simulink model "ASM_Traffic_new"  (R2024a)
settings: Solver=ode1  StartTime=SIM.tstart.v  StopTime=SIM.tend.v  FixedStep=SIM.StepSize.v  RelTol=1e-3
PostLoadFcn:
  | if any(exist('dsrtsu_mdlpostloadfcn', 'file') ~= 0), dsrtsu_mdlpostloadfcn('Execute', bdroot); end
  | try, asm_mdl_postloadfcn(bdroot, 'UpdateModel', 3600); catch, disp(lasterr); end,
InitFcn:
  | , if any(exist('rtifpga_mdlclblib', 'file') ~= 0), rtifpga_mdlclblib('Init', bdroot); end,
  | , if any(exist('dsmpb_private', 'file') ~= 0), dsmpb_private('dsmpb_mdlclblib', 'Init', bdroot); end,
undefined symbols (not defined in the file): _to_, a0b2, ASM_BrakeHydraulics_DemoSystems, ASM_VehicleDynamics_DemoSystems, b98103fe8ad365046cd0, BrakeCircuit, CPT, Crankshaft, DiscIntNeverNeededParam, dsmsi, FinalDriveAssembly, MDL, ModeSignals, Pos_BrakePedal_Maneuver, rad, RefSignals, s_to_rpm, SIM, SoftECU, Suspension, Tire, Transmission
libraries: ASM_Traffic_lib x135, simulink x100, ASM_Utils_lib x77, ASM_VehicleDynamics_lib x70, ASM_Environment_lib x22, dsmpblib x20, dsmsilib x15, MDLD_Utils_lib x10, ASM_BrakeHydraulics_lib x3
(part 22 of 63)

== system ASM_Traffic_new/Engine/Interface_In/ModelSignals/Reset_States[0|1]_ ==
  In1 : Inport
  Gain : Gain  SaturateOnIntegerOverflow=on  OutDataTypeStr=Inherit: Same as input  ParamDataTypeStr=Inherit: Same as input
  Out1 : Outport  VectorParamsAs1DForOutWhenUnconnected=off
  wires:
  In1/1 -> Gain/1
  Gain/1 -> Out1/1

== system ASM_Traffic_new/Engine/Interface_In/ModelSignals/State_StartButton[-1|0|1|2]_ ==
  In1 : Inport
  Gain : Gain  SaturateOnIntegerOverflow=on  OutDataTypeStr=Inherit: Same as input  ParamDataTypeStr=Inherit: Same as input
  Out1 : Outport  VectorParamsAs1DForOutWhenUnconnected=off
  wires:
  Gain/1 -> Out1/1
  In1/1 -> Gain/1

== system ASM_Traffic_new/Engine/Interface_In/ModelSignals/Sw_CrankShaft_Reset[0Disabled|1Enabled]_ ==
  In1 : Inport
  Gain : Gain  SaturateOnIntegerOverflow=on  OutDataTypeStr=Inherit: Same as input  ParamDataTypeStr=Inherit: Same as input
  Out1 : Outport  VectorParamsAs1DForOutWhenUnconnected=off
  wires:
  In1/1 -> Gain/1
  Gain/1 -> Out1/1

== system ASM_Traffic_new/Engine/Interface_In/ModelSignals/Sw_Ignition[0Off|1On]_ ==
  In1 : Inport
  Gain : Gain  SaturateOnIntegerOverflow=on  OutDataTypeStr=Inherit: Same as input  ParamDataTypeStr=Inherit: Same as input
  Out1 : Outport  VectorParamsAs1DForOutWhenUnconnected=off
  wires:
  In1/1 -> Gain/1
  Gain/1 -> Out1/1

== system ASM_Traffic_new/Engine/Interface_In/ModelSignals/Sw_ModelDeskPlottingInterface[0Disabled|1Enabled]_ ==
  In1 : Inport
  Gain : Gain
  Out1 : Outport
  wires:
  Gain/1 -> Out1/1
  In1/1 -> Gain/1

== system ASM_Traffic_new/Engine/Interface_In/ModelSignals/Sw_ModelPortBlocks[0Disabled|1Enabled]_ ==
  In1 : Inport
  Gain : Gain
  Out1 : Outport
  wires:
  Gain/1 -> Out1/1
  In1/1 -> Gain/1

== system ASM_Traffic_new/Engine/Interface_In/ModelSignals/Sw_StarterReq[0Off|1On]_ ==
  In1 : Inport
  Gain : Gain  SaturateOnIntegerOverflow=on  OutDataTypeStr=Inherit: Same as input  ParamDataTypeStr=Inherit: Same as input
  Out1 : Outport  VectorParamsAs1DForOutWhenUnconnected=off
  wires:
  In1/1 -> Gain/1
  Gain/1 -> Out1/1

== system ASM_Traffic_new/Engine/Interface_In/ModelSignals/Trq_Decrease_Request_Fast_ESP[Nm]_ ==
  In1 : Inport
  Gain : Gain  SaturateOnIntegerOverflow=on  OutDataTypeStr=Inherit: Same as input  ParamDataTypeStr=Inherit: Same as input
  Out1 : Outport  VectorParamsAs1DForOutWhenUnconnected=off
  wires:
  In1/1 -> Gain/1
  Gain/1 -> Out1/1

== system ASM_Traffic_new/Engine/Interface_In/ModelSignals/Trq_Increase_Request_Fast_ESP[Nm]_ ==
  In1 : Inport
  Gain : Gain  SaturateOnIntegerOverflow=on  OutDataTypeStr=Inherit: Same as input  ParamDataTypeStr=Inherit: Same as input
  Out1 : Outport  VectorParamsAs1DForOutWhenUnconnected=off
  wires:
  In1/1 -> Gain/1
  Gain/1 -> Out1/1

== system ASM_Traffic_new/Engine/Interface_In/ModelSignals/Trq_Request_Extern1[Nm]_ ==
  In1 : Inport
  Gain : Gain  SaturateOnIntegerOverflow=on  OutDataTypeStr=Inherit: Same as input  ParamDataTypeStr=Inherit: Same as input
  Out1 : Outport  VectorParamsAs1DForOutWhenUnconnected=off
  wires:
  In1/1 -> Gain/1
  Gain/1 -> Out1/1

== system ASM_Traffic_new/Engine/Interface_In/ModelSignals/Trq_Request_Extern2[Nm]_ ==
  In1 : Inport
  Gain : Gain  SaturateOnIntegerOverflow=on  OutDataTypeStr=Inherit: Same as input  ParamDataTypeStr=Inherit: Same as input
  Out1 : Outport  VectorParamsAs1DForOutWhenUnconnected=off
  wires:
  In1/1 -> Gain/1
  Gain/1 -> Out1/1

== system ASM_Traffic_new/Engine/Interface_In/ModelSignals/Trq_Request_ICE[Nm]_ ==
  In1 : Inport
  Gain : Gain  SaturateOnIntegerOverflow=on  OutDataTypeStr=Inherit: Same as input  ParamDataTypeStr=Inherit: Same as input
  Out1 : Outport  VectorParamsAs1DForOutWhenUnconnected=off
  wires:
  In1/1 -> Gain/1
  Gain/1 -> Out1/1

== system ASM_Traffic_new/Engine/Interface_In/ModelSignals/Vehicle_Topology[-2|-1|0|2]_ ==
  In1 : Inport
  Gain : Gain  SaturateOnIntegerOverflow=on  OutDataTypeStr=Inherit: Same as input  ParamDataTypeStr=Inherit: Same as input
  Out1 : Outport  VectorParamsAs1DForOutWhenUnconnected=off
  wires:
  In1/1 -> Gain/1
  Gain/1 -> Out1/1

== system ASM_Traffic_new/Engine/Interface_In/ModelSignals/n_Engine[rpm]_ ==
  In1 : Inport
  Gain : Gain  SaturateOnIntegerOverflow=on  OutDataTypeStr=Inherit: Same as input  ParamDataTypeStr=Inherit: Same as input
  Out1 : Outport  VectorParamsAs1DForOutWhenUnconnected=off
  wires:
  In1/1 -> Gain/1
  Gain/1 -> Out1/1

== system ASM_Traffic_new/Engine/Interface_In/ModelSignals/n_Engine_Idle_Request[rpm]_ ==
  In1 : Inport
  Gain : Gain  SaturateOnIntegerOverflow=on  OutDataTypeStr=Inherit: Same as input  ParamDataTypeStr=Inherit: Same as input
  Out1 : Outport  VectorParamsAs1DForOutWhenUnconnected=off
  wires:
  In1/1 -> Gain/1
  Gain/1 -> Out1/1

== system ASM_Traffic_new/Engine/Interface_In/ModelSignals/v_x_Vehicle[km|h]_ ==
  In1 : Inport
  Gain : Gain  SaturateOnIntegerOverflow=on  OutDataTypeStr=Inherit: Same as input  ParamDataTypeStr=Inherit: Same as input
  Out1 : Outport  VectorParamsAs1DForOutWhenUnconnected=off
  wires:
  In1/1 -> Gain/1
  Gain/1 -> Out1/1

== system ASM_Traffic_new/Engine/Interface_Out/Control_ModelSignals/CrankAngle_Cyl[aTDC]_ ==
  In1 : Inport
  DummyGain : Gain  SaturateOnIntegerOverflow=on  OutDataTypeStr=Inherit: Same as input  ParamDataTypeStr=Inherit: Same as input
  Out1 : Outport  VectorParamsAs1DForOutWhenUnconnected=off
  wires:
  DummyGain/1 -> Out1/1
  In1/1 -> DummyGain/1

== system ASM_Traffic_new/Engine/Interface_Out/Control_ModelSignals/Enable_Trq_Shift_Request[0|1]_ ==
  In1 : Inport
  Gain : Gain  SaturateOnIntegerOverflow=on  OutDataTypeStr=Inherit: Same as input  ParamDataTypeStr=Inherit: Same as input
  Out1 : Outport  VectorParamsAs1DForOutWhenUnconnected=off
  wires:
  Gain/1 -> Out1/1
  In1/1 -> Gain/1

== system ASM_Traffic_new/Engine/Interface_Out/Control_ModelSignals/EngOP_Num[]_ ==
  In1 : Inport
  DummyGain : Gain  SaturateOnIntegerOverflow=on  OutDataTypeStr=Inherit: Same as input  ParamDataTypeStr=Inherit: Same as input
  Out1 : Outport  VectorParamsAs1DForOutWhenUnconnected=off
  wires:
  In1/1 -> DummyGain/1
  DummyGain/1 -> Out1/1

== system ASM_Traffic_new/Engine/Interface_Out/Control_ModelSignals/Pos_AccPedal_Meas[%]_ ==
  In1 : Inport
  DummyGain : Gain  SaturateOnIntegerOverflow=on  OutDataTypeStr=Inherit: Same as input  ParamDataTypeStr=Inherit: Same as input
  Out1 : Outport  VectorParamsAs1DForOutWhenUnconnected=off
  wires:
  DummyGain/1 -> Out1/1
  In1/1 -> DummyGain/1

== system ASM_Traffic_new/Engine/Interface_Out/Control_ModelSignals/State_ICEngine[0|1|2|3|4]_ ==
  In1 : Inport
  Gain : Gain  SaturateOnIntegerOverflow=on  OutDataTypeStr=Inherit: Same as input  ParamDataTypeStr=Inherit: Same as input
  Out1 : Outport  VectorParamsAs1DForOutWhenUnconnected=off
  wires:
  In1/1 -> Gain/1
  Gain/1 -> Out1/1

== system ASM_Traffic_new/Engine/Interface_Out/Control_ModelSignals/State_StartStop[1Off|2NotReady|3Ready|4EngStopped]_ ==
  In1 : Inport
  Gain : Gain  SaturateOnIntegerOverflow=on  OutDataTypeStr=Inherit: Same as input  ParamDataTypeStr=Inherit: Same as input
  Out1 : Outport  VectorParamsAs1DForOutWhenUnconnected=off
  wires:
  In1/1 -> Gain/1
  Gain/1 -> Out1/1

== system ASM_Traffic_new/Engine/Interface_Out/Control_ModelSignals/Sw_Replace_Env[0|1]_ ==
  In1 : Inport
  DummyGain : Gain  SaturateOnIntegerOverflow=on  OutDataTypeStr=Inherit: Same as input  ParamDataTypeStr=Inherit: Same as input
  Out1 : Outport  VectorParamsAs1DForOutWhenUnconnected=off
  wires:
  DummyGain/1 -> Out1/1
  In1/1 -> DummyGain/1

== system ASM_Traffic_new/Engine/Interface_Out/Control_ModelSignals/Sw_Starter[0Off|1On]_ ==
  In1 : Inport
  Gain : Gain  SaturateOnIntegerOverflow=on  OutDataTypeStr=Inherit: Same as input  ParamDataTypeStr=Inherit: Same as input
  Out1 : Outport  VectorParamsAs1DForOutWhenUnconnected=off
  wires:
  In1/1 -> Gain/1
  Gain/1 -> Out1/1

== system ASM_Traffic_new/Engine/Interface_Out/Control_ModelSignals/T_Ambient[degC]_ ==
  In1 : Inport
  DummyGain : Gain  SaturateOnIntegerOverflow=on  OutDataTypeStr=Inherit: Same as input  ParamDataTypeStr=Inherit: Same as input
  Out1 : Outport  VectorParamsAs1DForOutWhenUnconnected=off
  wires:
  DummyGain/1 -> Out1/1
  In1/1 -> DummyGain/1

== system ASM_Traffic_new/Engine/Interface_Out/Control_ModelSignals/Trq_MeanEff_Engine_Meas[Nm]_ ==
  In1 : Inport
  DummyGain : Gain  SaturateOnIntegerOverflow=on  OutDataTypeStr=Inherit: Same as input  ParamDataTypeStr=Inherit: Same as input
  Out1 : Outport  VectorParamsAs1DForOutWhenUnconnected=off
  wires:
  DummyGain/1 -> Out1/1
  In1/1 -> DummyGain/1

== system ASM_Traffic_new/Engine/Interface_Out/Control_ModelSignals/Trq_Shift_Request[Nm]_ ==
  In1 : Inport
  Gain : Gain  SaturateOnIntegerOverflow=on  OutDataTypeStr=Inherit: Same as input  ParamDataTypeStr=Inherit: Same as input
  Out1 : Outport  VectorParamsAs1DForOutWhenUnconnected=off
  wires:
  In1/1 -> Gain/1
  Gain/1 -> Out1/1

== system ASM_Traffic_new/Engine/Interface_Out/Control_ModelSignals/n_Engine_Idle_Set[rpm]_ ==
  In1 : Inport
  Gain : Gain  SaturateOnIntegerOverflow=on  OutDataTypeStr=Inherit: Same as input  ParamDataTypeStr=Inherit: Same as input
  Out1 : Outport  VectorParamsAs1DForOutWhenUnconnected=off
  wires:
  In1/1 -> Gain/1
  Gain/1 -> Out1/1

== system ASM_Traffic_new/Engine/Interface_Out/Control_ModelSignals/n_Engine_Meas[rpm]_ ==
  In1 : Inport
  DummyGain : Gain  SaturateOnIntegerOverflow=on  OutDataTypeStr=Inherit: Same as input  ParamDataTypeStr=Inherit: Same as input
  Out1 : Outport  VectorParamsAs1DForOutWhenUnconnected=off
  wires:
  In1/1 -> DummyGain/1
  DummyGain/1 -> Out1/1

== system ASM_Traffic_new/Engine/Interface_Out/Control_ModelSignals/p_Ambient[Pa]_ ==
  In1 : Inport
  DummyGain : Gain  SaturateOnIntegerOverflow=on  OutDataTypeStr=Inherit: Same as input  ParamDataTypeStr=Inherit: Same as input
  Out1 : Outport  VectorParamsAs1DForOutWhenUnconnected=off
  wires:
  In1/1 -> DummyGain/1
  DummyGain/1 -> Out1/1

== system ASM_Traffic_new/Engine/Interface_Out/Plant_ModelSignals/T_Coolant_ICE[degC]_ ==
  In1 : Inport
  Gain : Gain  SaturateOnIntegerOverflow=on  OutDataTypeStr=Inherit: Same as input  ParamDataTypeStr=Inherit: Same as input
  Out1 : Outport  VectorParamsAs1DForOutWhenUnconnected=off
  wires:
  Gain/1 -> Out1/1
  In1/1 -> Gain/1

== system ASM_Traffic_new/Engine/Interface_Out/Plant_ModelSignals/Trq_Fric_Engine[Nm]_ ==
  In1 : Inport
  Gain : Gain  SaturateOnIntegerOverflow=on  OutDataTypeStr=Inherit: Same as input  ParamDataTypeStr=Inherit: Same as input
  Out1 : Outport  VectorParamsAs1DForOutWhenUnconnected=off
  wires:
  In1/1 -> Gain/1
  Gain/1 -> Out1/1

== system ASM_Traffic_new/Engine/Interface_Out/Plant_ModelSignals/Trq_MeanEff_Engine[Nm]_ ==
  In1 : Inport
  Gain : Gain  SaturateOnIntegerOverflow=on  OutDataTypeStr=Inherit: Same as input  ParamDataTypeStr=Inherit: Same as input
  Out1 : Outport  VectorParamsAs1DForOutWhenUnconnected=off
  wires:
  In1/1 -> Gain/1
  Gain/1 -> Out1/1

== system ASM_Traffic_new/Engine/Interface_Out/Plant_ModelSignals/Type_Engine[0Unkown|1Other|2Otto|3Diesel|4Electric]_ ==
  In1 : Inport
  DummyGain : Gain  SaturateOnIntegerOverflow=on  OutDataTypeStr=Inherit: Same as input  ParamDataTypeStr=Inherit: Same as input
  Out1 : Outport  VectorParamsAs1DForOutWhenUnconnected=off
  wires:
  In1/1 -> DummyGain/1
  DummyGain/1 -> Out1/1

== system ASM_Traffic_new/Engine/Plant/EngineBasic/ASMSignalCollector ==
  BusCreator : BusCreator  Inputs=2
  ASMSIgnalBus : Outport  VectorParamsAs1DForOutWhenUnconnected=off
  wires:
  [ASMBUS_FUEL_CONSUMPTION] -> BusCreator/2
  BusCreator/1 -> ASMSIgnalBus/1  "Plant"
  [ASMBUS_ENGINE] -> BusCreator/1

== system ASM_Traffic_new/Engine/Plant/UserInterface/ASMSignalBus_Plant ==
  In : Inport
  Terminator_1 : Terminator
  tag scope: ASMBUS_Engine_Plant=global
  wires:
  [ASMBUS_Engine_Plant] -> Terminator_1/1
  In/1 -> [ASMBUS_Engine_Plant]  "Plant"

== system ASM_Traffic_new/Engine/Plant/UserInterface/DISP_Plant ==
  note: Dummy blocks for ControlDesk layout.
      | Might be replaced when simulating virtual vehicles.
  Interface_In : Inport
  In : Inport  Port=2
  Bus Selector1 : BusSelector  OutputSignals=Engine.Trq_Eff_Engine[Nm],Engine.Trq_Fric_Engine[Nm],Engine.Trq_Ind_Engine[Nm]
  Bus Selector10 : BusSelector  OutputSignals=FuelConsumption.CO2_Emission.CO2_Emission[kg|h],FuelConsumption.CO2_Emission.CO2_Emission_Total[kg],FuelConsumption.Fuel_Consumption[l|h],FuelConsumption.Fuel_Consumption_Total[l],FuelConsumption.mdot_Fuel[g|h],FuelConsumption.b_e[g|kWh],FuelConsumption.Efficiency.eta_Eff_Engine[0_1],FuelConsumption.Efficiency.eta_Ind_Engine[0_1],FuelConsumption.Efficiency.eta_Mechanical_Engine[0_1]
  Bus Selector2 : BusSelector  OutputSignals=ExternalModel.v_x_Vehicle[km|h]
  CO2_Emission[kg|100km] : Subsystem
      mask Display: disp('')
  CO2_Emission[kg|100km]_ : Subsystem
  CO2_Emission[kg|h] : Subsystem
      mask Display: disp('')
  CO2_Emission_Total[kg] : Subsystem
      mask Display: disp('')
  CarbonEmission : Scope  NumInputPorts=3
  Efficiency : Scope  NumInputPorts=3
  Engine : Scope  NumInputPorts=3
  FuelConsumption : Scope  NumInputPorts=5
  FuelTank : Constant  Value=0.5
  FuelTank[0|1] : Subsystem
      mask Display: disp('')
  Fuel_Consumption[L|100km] : Subsystem
      mask Display: disp('')
  Fuel_Consumption[L|100km]_ : Subsystem
  Fuel_Consumption[l|h] : Subsystem
      mask Display: disp('')
  Fuel_Consumption_Total[l] : Subsystem
      mask Display: disp('')
  T_Water : Constant
  T_Water[degC] : Subsystem
      mask Display: disp('')
  Terminator : Terminator
  Terminator2 : Terminator
  Trq_Eff_Engine[Nm] : Subsystem
      mask Display: disp('')
  Trq_Fric_Engine[Nm] : Subsystem
      mask Display: disp('')
  Trq_Ind_Engine[Nm] : Subsystem
      mask Display: disp('')
  b_e[g|kWh] : Subsystem
      mask Display: disp('')
  eta_Eff_Engine[0_1] : Subsystem
      mask Display: disp('')
  eta_Ind_Engine[0_1] : Subsystem
      mask Display: disp('')
  eta_Mechanical_Engine[0_1] : Subsystem
      mask Display: disp('')
  mdot_Fuel[g|h] : Subsystem
      mask Display: disp('')
  wires:
  Bus Selector2/1 -> CO2_Emission[kg|100km]_/1(v_Vehicle[km|h]), Fuel_Consumption[L|100km]_/1(v_Vehicle[km|h])  "<v_x_Vehicle[km|h]>"
  Interface_In/1 -> Bus Selector2/1
  Bus Selector10/4 -> Fuel_Consumption_Total[l]/1(In1)  "<Fuel_Consumption_Total[l]>"
  T_Water[degC]/1(Out1) -> Terminator2/1
  FuelTank/1 -> FuelTank[0|1]/1(In1)
  Fuel_Consumption[L|100km]/1(Out1) -> FuelConsumption/1  "Fuel_Conumption[l|100km]"
  T_Water/1 -> T_Water[degC]/1(In1)
  FuelTank[0|1]/1(Out1) -> Terminator/1
  Trq_Ind_Engine[Nm]/1(Out1) -> Engine/3  "Trq_Ind_Engine[Nm]"
  Bus Selector1/1 -> Trq_Eff_Engine[Nm]/1(In1)  "<Trq_Eff_Engine[Nm]>"
  Fuel_Consumption[L|100km]_/1(Fuel_Consumption[L|100km]) -> Fuel_Consumption[L|100km]/1(In1)
  Bus Selector1/3 -> Trq_Ind_Engine[Nm]/1(In1)  "<Trq_Ind_Engine[Nm]>"
  Trq_Fric_Engine[Nm]/1(Out1) -> Engine/2  "Trq_Fric_Engine[Nm]"
  CO2_Emission_Total[kg]/1(Out1) -> CarbonEmission/3  "CO2_Emission_Total[kg]"
  Bus Selector10/3 -> Fuel_Consumption[l|h]/1(In1), Fuel_Consumption[L|100km]_/2(Fuel_Consumption[l|h])  "<Fuel_Consumption[l|h]>"
  Bus Selector1/2 -> Trq_Fric_Engine[Nm]/1(In1)  "<Trq_Fric_Engine[Nm]>"
  CO2_Emission[kg|100km]_/1(CO2_Emission[kg|100km]) -> CO2_Emission[kg|100km]/1(In1)
  eta_Eff_Engine[0_1]/1(Out1) -> Efficiency/1  "eta_Eff_Engine[0_1]"
  Bus Selector10/5 -> mdot_Fuel[g|h]/1(In1)  "<mdot_Fuel[g|h]>"
  Bus Selector10/1 -> CO2_Emission[kg|h]/1(In1), CO2_Emission[kg|100km]_/2(CO2_Emission[kg|h])  "<CO2_Emission[kg|h]>"
  Bus Selector10/6 -> b_e[g|kWh]/1(In1)  "<b_e[g|kWh]>"
  Bus Selector10/2 -> CO2_Emission_Total[kg]/1(In1)  "<CO2_Emission_Total[kg]>"
  Trq_Eff_Engine[Nm]/1(Out1) -> Engine/1  "Trq_Eff_Engine[Nm]"
  CO2_Emission[kg|h]/1(Out1) -> CarbonEmission/2  "CO2_Emission[kg|h]"
  Bus Selector10/7 -> eta_Eff_Engine[0_1]/1(In1)  "<eta_Eff_Engine[0_1]>"
  Fuel_Consumption_Total[l]/1(Out1) -> FuelConsumption/3  "Fuel_Consumption_Total[l]"
  Bus Selector10/9 -> eta_Mechanical_Engine[0_1]/1(In1)  "<eta_Mechanical_Engine[0_1]>"
  In/1 -> Bus Selector1/1, Bus Selector10/1
  Fuel_Consumption[l|h]/1(Out1) -> FuelConsumption/2  "Fuel_Consumption[l|h]"
  eta_Mechanical_Engine[0_1]/1(Out1) -> Efficiency/3  "eta_Mechanical_Engine[0_1]"
  Bus Selector10/8 -> eta_Ind_Engine[0_1]/1(In1)  "<eta_Ind_Engine[0_1]>"
  eta_Ind_Engine[0_1]/1(Out1) -> Efficiency/2  "eta_Ind_Engine[0_1]"
  CO2_Emission[kg|100km]/1(Out1) -> CarbonEmission/1  "CO2_Emission[kg|100km]"
  b_e[g|kWh]/1(Out1) -> FuelConsumption/5  "b_e[g|kWh]"
  mdot_Fuel[g|h]/1(Out1) -> FuelConsumption/4  "mdot_Fuel[g|h]"

== system ASM_Traffic_new/Engine/Plant/UserInterface/PAR_Plant ==
  Termination : Constant  Value=0
  Out : Outport  VectorParamsAs1DForOutWhenUnconnected=off
  wires:
  Termination/1 -> Out/1

== system ASM_Traffic_new/Engine/SignalInterface/ASMSignalInterface/signal_structure ==
  ASMSignalBus : Inport
  BusSelector_1 : BusSelector  OutputSignals=Control,Plant
  CO2_Emission : BusSelector  OutputSignals=CO2_Emission[kg|h],CO2_Emission_Total[kg]
  ContentID : Constant  Value=278498219
  Control : BusSelector  OutputSignals=ESP_Fast_Torque_Set,Shift_Torque_Set,Torque_Intervention,IdleSpeedControl,EngineOperation
  DataTypeConversion_2 : DataTypeConversion  OutDataTypeStr=double
  ESP_Fast_Torque_Set : BusSelector  OutputSignals=Sw_Engine_Dynamics_Fast[0|1],Enable_Trq_Request_Fast[0|1],Trq_Request_Fast[Nm]
  Efficiency : BusSelector  OutputSignals=eta_Eff_Engine[0_1],eta_Ind_Engine[0_1],eta_Mechanical_Engine[0_1]
  Engine : BusSelector  OutputSignals=TimeConst_Engine_Dynamics[s],Trq_Eff_Engine[Nm],Trq_Driver_Des[Nm],Trq_FullLoad_Engine[Nm],Trq_Fric_Engine[Nm],Trq_Ind_Engine[Nm],Trq_Driver_Ind_Des[Nm],Trq_Engine_Ind_Max[Nm]
  EngineOperation : BusSelector  OutputSignals=State_Engine[0|1|2|3|4],Sw_Starter[0Off|1On]
  FuelConsumption : BusSelector  OutputSignals=mdot_Fuel[g|h],b_e[g|kWh],Efficiency,CO2_Emission,Fuel_Consumption[l|h],Fuel_Consumption_Total[l]
  IdleSpeedControl : BusSelector  OutputSignals=n_Engine_Idle_Set[rpm],Pos_AccPedal_Ctrl[%]
  InfoBlock : Subsystem
      mask Display: fprintf('Structural changes of the signal bus require an update \nof the ''ASMSignalCollector'' block. \n\nTo start the update process double click the parent block.\n\n WARNING:\n During update this subsystem will be cleared completely')
  MDLD_DATA_CAPTURE : MDLD_Utils_lib/ModelDeskPlotInterface/DataCapture_Sfcn/MDLD_DATA_CAPTURE  inputPortWidth=41  measurementSignals=[0 0 0 0 0 0 0 0 0 0 0 0 0 0 0 0 0 0 0 0 0 0 0 0 0 0 0 0 0 0 0 0 0 0 0 0 0 0 0 0 0]  downsampling=1  samplingPeriod=SIM.StepSize.v  uuid=0  ASMProperties=struct('Name','mdld_data_capture','Version','1.0','Library','mdld_utils_lib')  startTriggerDelay=0  startTriggerLogic=0  startTriggerCount=0  startTriggerConditions=[0,0,0,0,0,0,0,0,0]  stopTriggerDelay=0  stopTriggerLogic=0  stopTriggerCount=0  stopTriggerConditions=[0,0,0,0,0,0,0,0,0]  ContentID_RefStruct=278498219
  Plant : BusSelector  OutputSignals=Engine,FuelConsumption
  Shift_Torque_Set : BusSelector  OutputSignals=Trq_Driver_Ind_Des[Nm],Trq_Ind_Set[Nm],Enable_Trq_Ind_Set[0|1]
  SignalFilter : Mux  Inputs=41
  SignalFilterGain : Gain
  Terminator : Terminator
  Torque_Intervention : BusSelector  OutputSignals=Pos_AccPedal_Request[%],Enable_Trq_Request_Fast[0|1],Enable_Trq_Request_Extern1[0|1],Enable_Trq_Request_Extern2[0|1],Enable_Trq_Request_Extern3[0|1],Trq_Request_Fast[Nm],Trq_Request_Extern1[Nm],Trq_Request_Extern2[Nm],Trq_Request_Extern3[Nm],Pos_AccPedal_Request_Fast[%],Pos_AccPedal_Request_Extern1[%],Pos_AccPedal_Request_Extern2[%],Pos_AccPedal_Request_Extern3[%],Pos_AccPedal_Request_Driver[%]
  wires:
  ASMSignalBus/1 -> BusSelector_1/1
  BusSelector_1/1 -> Control/1  "<Control>"
  Control/1 -> ESP_Fast_Torque_Set/1  "<ESP_Fast_Torque_Set>"
  Control/2 -> Shift_Torque_Set/1  "<Shift_Torque_Set>"
  Control/3 -> Torque_Intervention/1  "<Torque_Intervention>"
  Control/4 -> IdleSpeedControl/1  "<IdleSpeedControl>"
  Control/5 -> EngineOperation/1  "<EngineOperation>"
  BusSelector_1/2 -> Plant/1  "<Plant>"
  Plant/1 -> Engine/1  "<Engine>"
  Plant/2 -> FuelConsumption/1  "<FuelConsumption>"
  FuelConsumption/3 -> Efficiency/1  "<Efficiency>"
  FuelConsumption/4 -> CO2_Emission/1  "<CO2_Emission>"
  ContentID/1 -> Terminator/1
  ESP_Fast_Torque_Set/1 -> SignalFilter/1  "<Sw_Engine_Dynamics_Fast[0|1]>"
  ESP_Fast_Torque_Set/2 -> DataTypeConversion_2/1  "<Enable_Trq_Request_Fast[0|1]>"
  DataTypeConversion_2/1 -> SignalFilter/2
  ESP_Fast_Torque_Set/3 -> SignalFilter/3  "<Trq_Request_Fast[Nm]>"
  Shift_Torque_Set/1 -> SignalFilter/4  "<Trq_Driver_Ind_Des[Nm]>"
  Shift_Torque_Set/2 -> SignalFilter/5  "<Trq_Ind_Set[Nm]>"
  Shift_Torque_Set/3 -> SignalFilter/6  "<Enable_Trq_Ind_Set[0|1]>"
  Torque_Intervention/1 -> SignalFilter/7  "<Pos_AccPedal_Request[%]>"
  Torque_Intervention/2 -> SignalFilter/8  "<Enable_Trq_Request_Fast[0|1]>"
  Torque_Intervention/3 -> SignalFilter/9  "<Enable_Trq_Request_Extern1[0|1]>"
  Torque_Intervention/4 -> SignalFilter/10  "<Enable_Trq_Request_Extern2[0|1]>"
  Torque_Intervention/5 -> SignalFilter/11  "<Enable_Trq_Request_Extern3[0|1]>"
  Torque_Intervention/6 -> SignalFilter/12  "<Trq_Request_Fast[Nm]>"
  Torque_Intervention/7 -> SignalFilter/13  "<Trq_Request_Extern1[Nm]>"
  Torque_Intervention/8 -> SignalFilter/14  "<Trq_Request_Extern2[Nm]>"
  Torque_Intervention/9 -> SignalFilter/15  "<Trq_Request_Extern3[Nm]>"
  Torque_Intervention/10 -> SignalFilter/16  "<Pos_AccPedal_Request_Fast[%]>"
  Torque_Intervention/11 -> SignalFilter/17  "<Pos_AccPedal_Request_Extern1[%]>"
  Torque_Intervention/12 -> SignalFilter/18  "<Pos_AccPedal_Request_Extern2[%]>"
  Torque_Intervention/13 -> SignalFilter/19  "<Pos_AccPedal_Request_Extern3[%]>"
  Torque_Intervention/14 -> SignalFilter/20  "<Pos_AccPedal_Request_Driver[%]>"
  IdleSpeedControl/1 -> SignalFilter/21  "<n_Engine_Idle_Set[rpm]>"
  IdleSpeedControl/2 -> SignalFilter/22  "<Pos_AccPedal_Ctrl[%]>"
  EngineOperation/1 -> SignalFilter/23  "<State_Engine[0|1|2|3|4]>"
  EngineOperation/2 -> SignalFilter/24  "<Sw_Starter[0Off|1On]>"
  Engine/1 -> SignalFilter/25  "<TimeConst_Engine_Dynamics[s]>"
  Engine/2 -> SignalFilter/26  "<Trq_Eff_Engine[Nm]>"
  Engine/3 -> SignalFilter/27  "<Trq_Driver_Des[Nm]>"
  Engine/4 -> SignalFilter/28  "<Trq_FullLoad_Engine[Nm]>"
  Engine/5 -> SignalFilter/29  "<Trq_Fric_Engine[Nm]>"
  Engine/6 -> SignalFilter/30  "<Trq_Ind_Engine[Nm]>"
  Engine/7 -> SignalFilter/31  "<Trq_Driver_Ind_Des[Nm]>"
  Engine/8 -> SignalFilter/32  "<Trq_Engine_Ind_Max[Nm]>"
  FuelConsumption/1 -> SignalFilter/33  "<mdot_Fuel[g|h]>"
  FuelConsumption/2 -> SignalFilter/34  "<b_e[g|kWh]>"
  Efficiency/1 -> SignalFilter/35  "<eta_Eff_Engine[0_1]>"
  Efficiency/2 -> SignalFilter/36  "<eta_Ind_Engine[0_1]>"
  Efficiency/3 -> SignalFilter/37  "<eta_Mechanical_Engine[0_1]>"
  CO2_Emission/1 -> SignalFilter/38  "<CO2_Emission[kg|h]>"
  CO2_Emission/2 -> SignalFilter/39  "<CO2_Emission_Total[kg]>"
  FuelConsumption/5 -> SignalFilter/40  "<Fuel_Consumption[l|h]>"
  FuelConsumption/6 -> SignalFilter/41  "<Fuel_Consumption_Total[l]>"
  SignalFilter/1 -> SignalFilterGain/1
  SignalFilterGain/1 -> MDLD_DATA_CAPTURE/1

== system ASM_Traffic_new/Engine/SignalInterface/ExternalOutports/Select_Outport_Signals ==
  ASMSignalBus : Inport
  Bus Selector : BusSelector  OutputSignals=Plant.Engine,Plant.FuelConsumption
  Engine : Outport  VectorParamsAs1DForOutWhenUnconnected=off
  FuelConsumption : Outport  Port=2  VectorParamsAs1DForOutWhenUnconnected=off
  wires:
  ASMSignalBus/1 -> Bus Selector/1
  Bus Selector/1 -> Engine/1  "<Engine>"
  Bus Selector/2 -> FuelConsumption/1  "<FuelConsumption>"

== system ASM_Traffic_new/Environment/GroundTruth/PlantModel/Add_Time ==
  TimeSignal[s] : Inport
  Environmental_Conditions[] : Inport  Port=2
  Add : Sum
  Add1 : Sum
  Mux : Mux  Inputs=3
  Reset_Time : Subsystem
  Rounding Function : Rounding
  Saturation1 : Saturate  UpperLimit=inf  LowerLimit=0
  Selector : Selector  InputPortWidth=8  IndexOptions=Index vector (dialog)  Indices=7  OutputSizes=1
  Selector1 : Selector  InputPortWidth=8  IndexOptions=Index vector (dialog)  Indices=8  OutputSizes=1
  Selector2 : Selector  InputPortWidth=8  IndexOptions=Index vector (dialog)  Indices=(1:6)  OutputSizes=1
  EnvironmentConditions_Out[] : Outport  VectorParamsAs1DForOutWhenUnconnected=off
  wires:
  Mux/1 -> EnvironmentConditions_Out[]/1
  Selector2/1 -> Mux/1  "Environment_Signals_Rest[]"
  Reset_Time/1(Seconds_Out[s]) -> Mux/2  "Seconds_Since_Midnight[s]"
  Saturation1/1 -> Mux/3  "Unix_Timestamp[s]"
  Add/1 -> Saturation1/1
  Add1/1 -> Reset_Time/1(Seconds_In[s])
  Rounding Function/1 -> Add/1, Add1/1
  TimeSignal[s]/1 -> Rounding Function/1
  Selector1/1 -> Add/2  "Start_Unix_Timestamp[s]"
  Selector/1 -> Add1/2  "Start_Seconds_Since_Midnight[s]"
  Environmental_Conditions[]/1 -> Selector/1, Selector2/1, Selector1/1

== system ASM_Traffic_new/Environment/GroundTruth/PlantModel/AutomatedDrivingFunction[] ==
  In : Inport
  Bus Selector23 : BusSelector  OutputSignals=AutomatedDrivingFunction_ACC[],AutomatedDrivingFunction_AEB[],AutomatedDrivingFunction_FCW[],AutomatedDrivingFunction_4[]
  Bus_Selector_AutomatedDrivingFunction_4 : BusSelector  OutputSignals=Driver_Override_Active[0Off|1On],Driver_Override_Reason_Idx[],State_Idx[],Name_Idx[],Custom_Name_Idx[],Custom_State_Idx[],Key_1_Idx[],Value_1_Idx[],Key_2_Idx[],Value_2_Idx[]
  Bus_Selector_AutomatedDrivingFunction_ACC : BusSelector  OutputSignals=Driver_Override_Active[0Off|1On],Driver_Override_Reason_Idx[],State_Idx[],Name_Idx[],Custom_Name_Idx[],Custom_State_Idx[],Key_1_Idx[],Value_1_Idx[],Key_2_Idx[],Value_2_Idx[]
  Bus_Selector_AutomatedDrivingFunction_AEB : BusSelector  OutputSignals=Driver_Override_Reason_Idx[],Driver_Override_Reason_Idx[],State_Idx[],Name_Idx[],Custom_Name_Idx[],Custom_State_Idx[],Key_1_Idx[],Value_1_Idx[],Key_2_Idx[],Value_2_Idx[]
  Bus_Selector_AutomatedDrivingFunction_FCW : BusSelector  OutputSignals=Driver_Override_Active[0Off|1On],Driver_Override_Reason_Idx[],State_Idx[],Name_Idx[],Custom_Name_Idx[],Custom_State_Idx[],Key_1_Idx[],Value_1_Idx[],Key_2_Idx[],Value_2_Idx[]
  Mux4 : Mux
  Mux_AutomatedDrivingFunction_4 : Mux  Inputs=10
  Mux_AutomatedDrivingFunction_ACC : Mux  Inputs=10
  Mux_AutomatedDrivingFunction_AEB : Mux  Inputs=10
  Mux_AutomatedDrivingFunction_FCW : Mux  Inputs=10
  AutomatedDrivingFunction[] : Outport  VectorParamsAs1DForOutWhenUnconnected=off
  wires:
  In/1 -> Bus Selector23/1
  Bus Selector23/1 -> Bus_Selector_AutomatedDrivingFunction_ACC/1  "<AutomatedDrivingFunction_ACC[]>"
  Bus Selector23/2 -> Bus_Selector_AutomatedDrivingFunction_AEB/1  "<AutomatedDrivingFunction_AEB[]>"
  Bus Selector23/3 -> Bus_Selector_AutomatedDrivingFunction_FCW/1  "<AutomatedDrivingFunction_FCW[]>"
  Bus Selector23/4 -> Bus_Selector_AutomatedDrivingFunction_4/1  "<AutomatedDrivingFunction_4[]>"
  Bus_Selector_AutomatedDrivingFunction_ACC/1 -> Mux_AutomatedDrivingFunction_ACC/1  "<Driver_Override_Active[0Off|1On]>"
  Bus_Selector_AutomatedDrivingFunction_ACC/2 -> Mux_AutomatedDrivingFunction_ACC/2  "<Driver_Override_Reason_Idx[]>"
  Bus_Selector_AutomatedDrivingFunction_ACC/3 -> Mux_AutomatedDrivingFunction_ACC/3  "<State_Idx[]>"
  Bus_Selector_AutomatedDrivingFunction_ACC/4 -> Mux_AutomatedDrivingFunction_ACC/4  "<Name_Idx[]>"
  Bus_Selector_AutomatedDrivingFunction_ACC/5 -> Mux_AutomatedDrivingFunction_ACC/5  "<Custom_Name_Idx[]>"
  Bus_Selector_AutomatedDrivingFunction_ACC/6 -> Mux_AutomatedDrivingFunction_ACC/6  "<Custom_State_Idx[]>"
  Bus_Selector_AutomatedDrivingFunction_ACC/7 -> Mux_AutomatedDrivingFunction_ACC/7  "<Key_1_Idx[]>"
  Bus_Selector_AutomatedDrivingFunction_ACC/8 -> Mux_AutomatedDrivingFunction_ACC/8  "<Value_1_Idx[]>"
  Bus_Selector_AutomatedDrivingFunction_ACC/9 -> Mux_AutomatedDrivingFunction_ACC/9  "<Key_2_Idx[]>"
  Bus_Selector_AutomatedDrivingFunction_ACC/10 -> Mux_AutomatedDrivingFunction_ACC/10  "<Value_2_Idx[]>"
  Bus_Selector_AutomatedDrivingFunction_AEB/1 -> Mux_AutomatedDrivingFunction_AEB/1  "<Driver_Override_Reason_Idx[]>"
  Bus_Selector_AutomatedDrivingFunction_AEB/2 -> Mux_AutomatedDrivingFunction_AEB/2  "<Driver_Override_Reason_Idx[]>"
  Bus_Selector_AutomatedDrivingFunction_AEB/3 -> Mux_AutomatedDrivingFunction_AEB/3  "<State_Idx[]>"
  Bus_Selector_AutomatedDrivingFunction_AEB/4 -> Mux_AutomatedDrivingFunction_AEB/4  "<Name_Idx[]>"
  Bus_Selector_AutomatedDrivingFunction_AEB/5 -> Mux_AutomatedDrivingFunction_AEB/5  "<Custom_Name_Idx[]>"
  Bus_Selector_AutomatedDrivingFunction_AEB/6 -> Mux_AutomatedDrivingFunction_AEB/6  "<Custom_State_Idx[]>"
  Bus_Selector_AutomatedDrivingFunction_AEB/7 -> Mux_AutomatedDrivingFunction_AEB/7  "<Key_1_Idx[]>"
  Bus_Selector_AutomatedDrivingFunction_AEB/8 -> Mux_AutomatedDrivingFunction_AEB/8  "<Value_1_Idx[]>"
  Bus_Selector_AutomatedDrivingFunction_AEB/9 -> Mux_AutomatedDrivingFunction_AEB/9  "<Key_2_Idx[]>"
  Bus_Selector_AutomatedDrivingFunction_AEB/10 -> Mux_AutomatedDrivingFunction_AEB/10  "<Value_2_Idx[]>"
  Bus_Selector_AutomatedDrivingFunction_FCW/1 -> Mux_AutomatedDrivingFunction_FCW/1  "<Driver_Override_Active[0Off|1On]>"
  Bus_Selector_AutomatedDrivingFunction_FCW/2 -> Mux_AutomatedDrivingFunction_FCW/2  "<Driver_Override_Reason_Idx[]>"
  Bus_Selector_AutomatedDrivingFunction_FCW/3 -> Mux_AutomatedDrivingFunction_FCW/3  "<State_Idx[]>"
  Bus_Selector_AutomatedDrivingFunction_FCW/4 -> Mux_AutomatedDrivingFunction_FCW/4  "<Name_Idx[]>"
  Bus_Selector_AutomatedDrivingFunction_FCW/5 -> Mux_AutomatedDrivingFunction_FCW/5  "<Custom_Name_Idx[]>"
  Bus_Selector_AutomatedDrivingFunction_FCW/6 -> Mux_AutomatedDrivingFunction_FCW/6  "<Custom_State_Idx[]>"
  Bus_Selector_AutomatedDrivingFunction_FCW/7 -> Mux_AutomatedDrivingFunction_FCW/7  "<Key_1_Idx[]>"
  Bus_Selector_AutomatedDrivingFunction_FCW/8 -> Mux_AutomatedDrivingFunction_FCW/8  "<Value_1_Idx[]>"
  Bus_Selector_AutomatedDrivingFunction_FCW/9 -> Mux_AutomatedDrivingFunction_FCW/9  "<Key_2_Idx[]>"
  Bus_Selector_AutomatedDrivingFunction_FCW/10 -> Mux_AutomatedDrivingFunction_FCW/10  "<Value_2_Idx[]>"
  Bus_Selector_AutomatedDrivingFunction_4/1 -> Mux_AutomatedDrivingFunction_4/1  "<Driver_Override_Active[0Off|1On]>"
  Bus_Selector_AutomatedDrivingFunction_4/2 -> Mux_AutomatedDrivingFunction_4/2  "<Driver_Override_Reason_Idx[]>"
  Bus_Selector_AutomatedDrivingFunction_4/3 -> Mux_AutomatedDrivingFunction_4/3  "<State_Idx[]>"
  Bus_Selector_AutomatedDrivingFunction_4/4 -> Mux_AutomatedDrivingFunction_4/4  "<Name_Idx[]>"
  Bus_Selector_AutomatedDrivingFunction_4/5 -> Mux_AutomatedDrivingFunction_4/5  "<Custom_Name_Idx[]>"
  Bus_Selector_AutomatedDrivingFunction_4/6 -> Mux_AutomatedDrivingFunction_4/6  "<Custom_State_Idx[]>"
  Bus_Selector_AutomatedDrivingFunction_4/7 -> Mux_AutomatedDrivingFunction_4/7  "<Key_1_Idx[]>"
  Bus_Selector_AutomatedDrivingFunction_4/8 -> Mux_AutomatedDrivingFunction_4/8  "<Value_1_Idx[]>"
  Bus_Selector_AutomatedDrivingFunction_4/9 -> Mux_AutomatedDrivingFunction_4/9  "<Key_2_Idx[]>"
  Bus_Selector_AutomatedDrivingFunction_4/10 -> Mux_AutomatedDrivingFunction_4/10  "<Value_2_Idx[]>"
  Mux_AutomatedDrivingFunction_ACC/1 -> Mux4/1
  Mux_AutomatedDrivingFunction_AEB/1 -> Mux4/2
  Mux_AutomatedDrivingFunction_FCW/1 -> Mux4/3
  Mux_AutomatedDrivingFunction_4/1 -> Mux4/4
  Mux4/1 -> AutomatedDrivingFunction[]/1

== system ASM_Traffic_new/Environment/GroundTruth/PlantModel/GetFellowPositionVector ==
  FellowPositions : Inport
  Bus Selector11 : BusSelector  OutputSignals=Pos_Fellows_MainPnt_CoorSys_E[x;y;z][m].Pos_x_Fellows[m],Pos_Fellows_MainPnt_CoorSys_E[x;y;z][m].Pos_y_Fellows[m],Pos_Fellows_MainPnt_CoorSys_E[x;y;z][m].Pos_z_Fellows[m],Angle_Fellows[x;y;z][deg].Angle_Roll_Fellows[deg],Angle_Fellows[x;y;z][deg].Angle_Pitch_Fellows[deg],Angle_Fellows[x;y;z][deg].Angle_Yaw_Fellows[deg]
  Mux1 : Mux  Inputs=3
  Mux2 : Mux  Inputs=3
  Pos_Fellows_MainPnt_CoorSys_E[x;y;z][m] : Outport  VectorParamsAs1DForOutWhenUnconnected=off
  Angle_Fellows[deg] : Outport  Port=2  VectorParamsAs1DForOutWhenUnconnected=off
  wires:
  Mux2/1 -> Pos_Fellows_MainPnt_CoorSys_E[x;y;z][m]/1  "Pos_Fellows_MainPnt_CoorSys_E[x;y;z][m]"
  Mux1/1 -> Angle_Fellows[deg]/1  "Pos_Fellows_MainPnt_CoorSys_E_vec"
  Bus Selector11/4 -> Mux1/1  "<Angle_Roll_Fellows[deg]>"
  Bus Selector11/1 -> Mux2/1  "<Pos_x_Fellows[m]>"
  Bus Selector11/2 -> Mux2/2  "<Pos_y_Fellows[m]>"
  Bus Selector11/6 -> Mux1/3  "<Angle_Yaw_Fellows[deg]>"
  Bus Selector11/5 -> Mux1/2  "<Angle_Pitch_Fellows[deg]>"
  FellowPositions/1 -> Bus Selector11/1
  Bus Selector11/3 -> Mux2/3  "<Pos_z_Fellows[m]>"

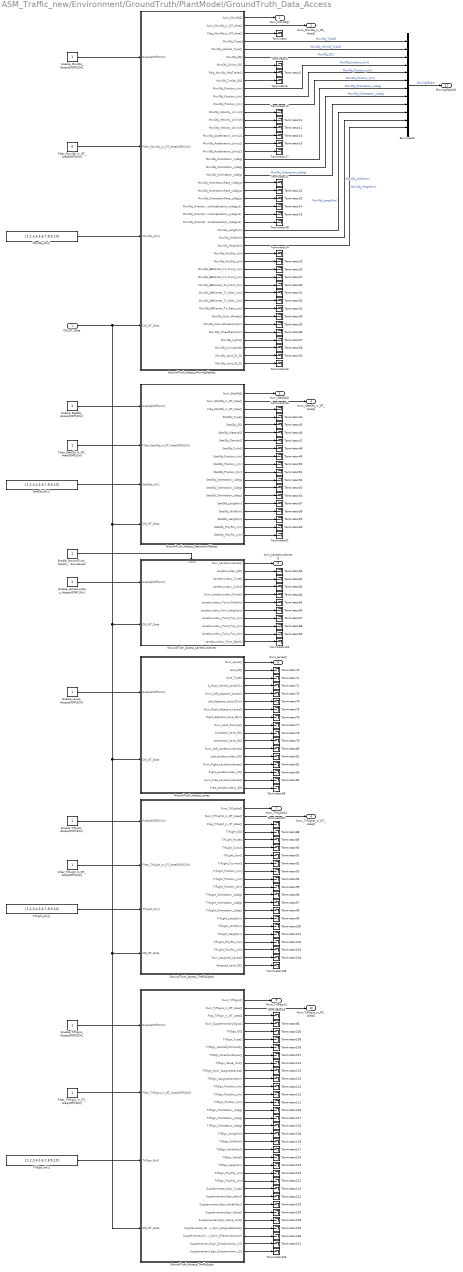
== system ASM_Traffic_new/Environment/GroundTruth/PlantModel/GroundTruth_Data_Access ==
  OSI_GT_Data : Inport
  Bus Creator : BusCreator  Inputs=12
  Enable_GroundTruth_Access_Laneboundaries : Constant
  Enable_Laneboundary_Access[0Off|1On] : Constant
  Enable_Lanes_Access[0Off|1On] : Constant
  Enable_MovObj_Access[0Off|1On] : Constant
  Enable_StatObj_Access[0Off|1On] : Constant
  Enable_TrfLight_Access[0Off|1On] : Constant
  Enable_TrfSigns_Access[0Off|1On] : Constant
  Filter_MovObj_In_GT_Area[0Off|1On] : Constant  Value=0
  Filter_StatObj_In_GT_Area[0Off|1On] : Constant
  Filter_TrfLight_In_GT_Area[0Off|1On] : Constant
  Filter_TrfSigns_In_GT_Area[0Off|1On] : Constant
  GroundTruth_Access_Laneboundaries : Subsystem
  GroundTruth_Access_Lanes : Subsystem
  GroundTruth_Access_MovingObjects : Subsystem
  GroundTruth_Access_StationaryObjects : Subsystem
  GroundTruth_Access_TrafficLights : Subsystem
  GroundTruth_Access_TrafficSigns : Subsystem
  MovObj_Idx[] : Constant  Value=[1,2,3,4,5,6,7,8,9,10]
  StatObj_Idx[] : Constant  Value=[1,2,3,4,5,6,7,8,9,10]
  Terminator{,4..6,10..17,21..38,42..133,135..136} (124 alike) : Terminator
  TrfLight_Idx[] : Constant  Value=[1,2,3,4,5,6,7,8,9,10]
  TrfSign_Idx[] : Constant  Value=[1,2,3,4,5,6,7,8,9,10]
  Num_MovObj[] : Outport  VectorParamsAs1DForOutWhenUnconnected=off
  Num_MovObj_in_GT_Area[] : Outport  Port=2  VectorParamsAs1DForOutWhenUnconnected=off
  Num_StatObj[] : Outport  Port=3  VectorParamsAs1DForOutWhenUnconnected=off
  Num_StatObj_in_GT_Area[] : Outport  Port=4  VectorParamsAs1DForOutWhenUnconnected=off
  Num_Laneboundaries[] : Outport  Port=5  VectorParamsAs1DForOutWhenUnconnected=off
  Num_Lanes[] : Outport  Port=6  VectorParamsAs1DForOutWhenUnconnected=off
  Num_TrfLights[] : Outport  Port=7  VectorParamsAs1DForOutWhenUnconnected=off
  Num_TrfLights_in_GT_Area[] : Outport  Port=8  VectorParamsAs1DForOutWhenUnconnected=off
  Num_TrfSigns[] : Outport  Port=9  VectorParamsAs1DForOutWhenUnconnected=off
  Num_TrfSigns_in_GT_Area[] : Outport  Port=10  VectorParamsAs1DForOutWhenUnconnected=off
  MovingObject[] : Outport  Port=11
  wires:
  Bus Creator/1 -> MovingObject[]/1  "MovingObject"
  GroundTruth_Access_Laneboundaries/11(Laneboundary_Point_Dash[]) -> Terminator132/1
  Enable_GroundTruth_Access_Laneboundaries/1 -> GroundTruth_Access_Laneboundaries/Enable
  GroundTruth_Access_MovingObjects/45(MovObj_Lane_ID_2[]) -> Terminator42/1
  GroundTruth_Access_MovingObjects/44(MovObj_Lane_ID_1[]) -> Terminator29/1
  GroundTruth_Access_MovingObjects/43(MovObj_NumLanes[]) -> Terminator28/1
  GroundTruth_Access_MovingObjects/42(MovObj_Lights[]) -> Terminator37/1
  GroundTruth_Access_MovingObjects/41(MovObj_WheelRadius[m]) -> Terminator36/1
  GroundTruth_Access_MovingObjects/40(MovObj_GroundClearance[m]) -> Terminator35/1
  GroundTruth_Access_MovingObjects/39(MovObj_Num_Wheels[]) -> Terminator34/1
  GroundTruth_Access_MovingObjects/38(MovObj_BBCenter_To_Rear_z[m]) -> Terminator33/1
  GroundTruth_Access_MovingObjects/37(MovObj_BBCenter_To_Rear_y[m]) -> Terminator32/1
  GroundTruth_Access_MovingObjects/36(MovObj_BBCenter_To_Rear_x[m]) -> Terminator31/1
  GroundTruth_Access_MovingObjects/35(MovObj_BBCenter_To_Front_z[m]) -> Terminator30/1
  GroundTruth_Access_MovingObjects/34(MovObj_BBCenter_To_Front_y[m]) -> Terminator27/1
  GroundTruth_Access_MovingObjects/33(MovObj_BBCenter_To_Front_x[m]) -> Terminator26/1
  GroundTruth_Access_MovingObjects/32(MovObj_PolyPts_y[m]) -> Terminator25/1
  GroundTruth_Access_MovingObjects/31(MovObj_PolyPts_x[m]) -> Terminator24/1
  GroundTruth_Access_MovingObjects/30(MovObj_Height[m]) -> Bus Creator/12  "MovObj_Height[m]"
  GroundTruth_Access_MovingObjects/29(MovObj_Width[m]) -> Bus Creator/11  "MovObj_Width[m]"
  GroundTruth_Access_MovingObjects/28(MovObj_Length[m]) -> Bus Creator/10  "MovObj_Length[m]"
  GroundTruth_Access_MovingObjects/27(MovObj_OrientationAcceleration_z[deg|s2]) -> Terminator38/1
  GroundTruth_Access_MovingObjects/26(MovObj_OrientationAcceleration_y[deg|s2]) -> Terminator15/1
  GroundTruth_Access_MovingObjects/25(MovObj_OrientationAcceleration_x[deg|s2]) -> Terminator14/1
  GroundTruth_Access_MovingObjects/24(MovObj_OrientationRate_z[deg|s]) -> Terminator23/1
  GroundTruth_Access_MovingObjects/23(MovObj_OrientationRate_y[deg|s]) -> Terminator22/1
  GroundTruth_Access_MovingObjects/22(MovObj_OrientationRate_x[deg|s]) -> Terminator21/1
  GroundTruth_Access_MovingObjects/21(MovObj_Orientation_z[deg]) -> Bus Creator/9  "MovObj_Orientation_z[deg]"
  GroundTruth_Access_MovingObjects/20(MovObj_Orientation_y[deg]) -> Bus Creator/8  "MovObj_Orientation_y[deg]"
  GroundTruth_Access_MovingObjects/19(MovObj_Orientation_x[deg]) -> Bus Creator/7  "MovObj_Orientation_x[deg]"
  GroundTruth_Access_MovingObjects/18(MovObj_Acceleration_z[m|s2]) -> Terminator17/1
  GroundTruth_Access_MovingObjects/17(MovObj_Acceleration_y[m|s2]) -> Terminator16/1
  GroundTruth_Access_MovingObjects/16(MovObj_Acceleration_x[m|s2]) -> Terminator13/1
  GroundTruth_Access_MovingObjects/15(MovObj_Velocity_z[km|h]) -> Terminator12/1
  GroundTruth_Access_MovingObjects/14(MovObj_Velocity_y[km|h]) -> Terminator11/1
  GroundTruth_Access_MovingObjects/13(MovObj_Velocity_x[km|h]) -> Terminator10/1
  GroundTruth_Access_MovingObjects/12(MovObj_Position_z[m]) -> Bus Creator/6  "MovObj_Position_z[m]"
  GroundTruth_Access_MovingObjects/11(MovObj_Position_y[m]) -> Bus Creator/5  "MovObj_Position_y[m]"
  GroundTruth_Access_MovingObjects/10(MovObj_Position_x[m]) -> Bus Creator/4  "MovObj_Position_x[m]"
  GroundTruth_Access_MovingObjects/9(MovObj_Trailer_ID[]) -> Terminator6/1
  GroundTruth_Access_MovingObjects/8(Flag_MovObj_HasTrailer[]) -> Terminator5/1
  GroundTruth_Access_MovingObjects/7(MovObj_Driver_ID[]) -> Terminator4/1
  GroundTruth_Access_MovingObjects/6(MovObj_ID[]) -> Bus Creator/3  "MovObj_ID[]"
  GroundTruth_Access_MovingObjects/5(MovObj_Vehicle_Type[]) -> Bus Creator/2  "MovObj_Vehicle_Type[]"
  GroundTruth_Access_MovingObjects/4(MovObj_Type[]) -> Bus Creator/1  "MovObj_Type[]"
  GroundTruth_Access_MovingObjects/3(Flag_MovObj_in_GT_Area[]) -> Terminator/1
  GroundTruth_Access_MovingObjects/2(Num_MovObj_in_GT_Area[]) -> Num_MovObj_in_GT_Area[]/1
  GroundTruth_Access_MovingObjects/1(Num_MovObj[]) -> Num_MovObj[]/1
  OSI_GT_Data/1 -> GroundTruth_Access_StationaryObjects/4(OSI_GT_Data), GroundTruth_Access_TrafficSigns/4(OSI_GT_Data), GroundTruth_Access_TrafficLights/4(OSI_GT_Data), GroundTruth_Access_Lanes/2(OSI_GT_Data), GroundTruth_Access_Laneboundaries/2(OSI_GT_Data), GroundTruth_Access_MovingObjects/4(OSI_GT_Data)
  MovObj_Idx[]/1 -> GroundTruth_Access_MovingObjects/3(MovObj_Idx[])
  Filter_MovObj_In_GT_Area[0Off|1On]/1 -> GroundTruth_Access_MovingObjects/2(Filter_MovObj_In_GT_Area[0Off|1On])
  Enable_MovObj_Access[0Off|1On]/1 -> GroundTruth_Access_MovingObjects/1(Enable[0Off|1On])
  GroundTruth_Access_StationaryObjects/2(Num_StatObj_in_GT_Area[]) -> Num_StatObj_in_GT_Area[]/1
  Enable_StatObj_Access[0Off|1On]/1 -> GroundTruth_Access_StationaryObjects/1(Enable[0Off|1On])
  Filter_StatObj_In_GT_Area[0Off|1On]/1 -> GroundTruth_Access_StationaryObjects/2(Filter_StatObj_In_GT_Area[0Off|1On])
  StatObj_Idx[]/1 -> GroundTruth_Access_StationaryObjects/3(StatObj_Idx[])
  GroundTruth_Access_Laneboundaries/1(Num_Laneboundaries[]) -> Num_Laneboundaries[]/1
  GroundTruth_Access_Laneboundaries/2(Laneboundary_ID[]) -> Terminator56/1
  GroundTruth_Access_Laneboundaries/3(Laneboundary_Type[]) -> Terminator62/1
  GroundTruth_Access_Laneboundaries/4(Laneboundary_Color[]) -> Terminator63/1
  GroundTruth_Access_Laneboundaries/5(Num_Laneboundary_Points[]) -> Terminator64/1
  GroundTruth_Access_Laneboundaries/6(Laneboundary_Point_Width[m]) -> Terminator65/1
  GroundTruth_Access_Laneboundaries/7(Laneboundary_Point_Height[m]) -> Terminator66/1
  GroundTruth_Access_Laneboundaries/8(Laneboundary_Point_Pos_x[m]) -> Terminator67/1
  GroundTruth_Access_Laneboundaries/9(Laneboundary_Point_Pos_y[m]) -> Terminator68/1
  GroundTruth_Access_Laneboundaries/10(Laneboundary_Point_Pos_z[m]) -> Terminator69/1
  Enable_Laneboundary_Access[0Off|1On]/1 -> GroundTruth_Access_Laneboundaries/1(Enable[0Off|1On])
  GroundTruth_Access_Lanes/1(Num_Lanes[]) -> Num_Lanes[]/1
  GroundTruth_Access_Lanes/2(Lane_ID[]) -> Terminator70/1
  GroundTruth_Access_Lanes/3(Lane_Type[]) -> Terminator71/1
  GroundTruth_Access_Lanes/4(Is_Host_Vehicle_Lane[0|1]) -> Terminator72/1
  GroundTruth_Access_Lanes/5(Num_Left_Adjacent_Lanes[]) -> Terminator73/1
  GroundTruth_Access_Lanes/6(Left_Adjacent_Lane_ID[m]) -> Terminator74/1
  GroundTruth_Access_Lanes/7(Num_Right_Adjacent_Lanes[]) -> Terminator75/1
  GroundTruth_Access_Lanes/8(Right_Adjacent_Lane_ID[m]) -> Terminator76/1
  GroundTruth_Access_Lanes/9(Num_Lane_Pairings[]) -> Terminator77/1
  GroundTruth_Access_Lanes/10(Successor_Lane_ID[]) -> Terminator78/1
  GroundTruth_Access_Lanes/11(Antecessor_Lane_ID[]) -> Terminator79/1
  GroundTruth_Access_Lanes/12(Num_Left_Laneboundaries[]) -> Terminator80/1
  GroundTruth_Access_Lanes/13(Left_Laneboundary_ID[]) -> Terminator81/1
  GroundTruth_Access_Lanes/14(Num_Right_Laneboundaries[]) -> Terminator82/1
  GroundTruth_Access_Lanes/15(Right_Laneboundary_ID[]) -> Terminator83/1
  GroundTruth_Access_Lanes/16(Num_Free_Laneboundaries[]) -> Terminator84/1
  GroundTruth_Access_Lanes/17(Free_Laneboundary_ID[]) -> Terminator85/1
  Enable_Lanes_Access[0Off|1On]/1 -> GroundTruth_Access_Lanes/1(Enable[0Off|1On])
  GroundTruth_Access_TrafficLights/2(Num_TrfLights_in_GT_Area[]) -> Num_TrfLights_in_GT_Area[]/1
  GroundTruth_Access_TrafficLights/1(Num_TrfLights[]) -> Num_TrfLights[]/1
  GroundTruth_Access_TrafficLights/3(Flag_TrfLight_in_GT_Area[]) -> Terminator87/1
  GroundTruth_Access_TrafficLights/4(TrfLight_ID[]) -> Terminator88/1
  GroundTruth_Access_TrafficLights/5(TrfLight_Mode[]) -> Terminator89/1
  GroundTruth_Access_TrafficLights/6(TrfLight_Color[]) -> Terminator90/1
  GroundTruth_Access_TrafficLights/7(TrfLight_Icon[]) -> Terminator91/1
  GroundTruth_Access_TrafficLights/8(TrfLight_Counter[]) -> Terminator92/1
  GroundTruth_Access_TrafficLights/9(TrfLight_Position_x[m]) -> Terminator93/1
  GroundTruth_Access_TrafficLights/10(TrfLight_Position_y[m]) -> Terminator94/1
  GroundTruth_Access_TrafficLights/11(TrfLight_Position_z[m]) -> Terminator95/1
  GroundTruth_Access_TrafficLights/12(TrfLight_Orientation_x[deg]) -> Terminator96/1
  GroundTruth_Access_TrafficLights/13(TrfLight_Orientation_y[deg]) -> Terminator97/1
  GroundTruth_Access_TrafficLights/14(TrfLight_Orientation_z[deg]) -> Terminator98/1
  GroundTruth_Access_TrafficLights/15(TrfLight_Length[m]) -> Terminator99/1
  GroundTruth_Access_TrafficLights/16(TrfLight_Width[m]) -> Terminator100/1
  GroundTruth_Access_TrafficLights/17(TrfLight_Height[m]) -> Terminator101/1
  GroundTruth_Access_TrafficLights/18(TrfLight_PolyPts_x[m]) -> Terminator102/1
  GroundTruth_Access_TrafficLights/19(TrfLight_PolyPts_y[m]) -> Terminator103/1
  GroundTruth_Access_TrafficLights/20(Num_Assigned_Lanes[]) -> Terminator104/1
  GroundTruth_Access_TrafficLights/21(Assigned_Lane_ID[]) -> Terminator105/1
  Enable_TrfLight_Access[0Off|1On]/1 -> GroundTruth_Access_TrafficLights/1(Enable[0Off|1On])
  Filter_TrfLight_In_GT_Area[0Off|1On]/1 -> GroundTruth_Access_TrafficLights/2(Filter_TrfLight_In_GT_Area[0Off|1On])
  TrfLight_Idx[]/1 -> GroundTruth_Access_TrafficLights/3(TrfLight_Idx[])
  GroundTruth_Access_TrafficSigns/3(Flag_TrfSign_in_GT_Area[]) -> Terminator55/1
  GroundTruth_Access_TrafficSigns/4(Num_SupplementarySigns[]) -> Terminator86/1
  GroundTruth_Access_TrafficSigns/5(TrfSign_ID[]) -> Terminator106/1
  GroundTruth_Access_TrafficSigns/6(TrfSign_Type[]) -> Terminator108/1
  GroundTruth_Access_TrafficSigns/7(TrfSign_VerticallyMirrored[]) -> Terminator109/1
  GroundTruth_Access_TrafficSigns/8(TrfSign_DirectionScope[]) -> Terminator107/1
  GroundTruth_Access_TrafficSigns/14(TrfSign_Position_z[m]) -> Terminator111/1
  GroundTruth_Access_TrafficSigns/13(TrfSign_Position_y[m]) -> Terminator113/1
  GroundTruth_Access_TrafficSigns/12(TrfSign_Position_x[m]) -> Terminator112/1
  GroundTruth_Access_TrafficSigns/11(TrfSign_AssignedLanes[m]) -> Terminator110/1
  GroundTruth_Access_TrafficSigns/10(TrfSign_Num_AssignedLanes[]) -> Terminator115/1
  GroundTruth_Access_TrafficSigns/9(TrfSign_Value_Unit[]) -> Terminator114/1
  GroundTruth_Access_TrafficSigns/21(TrfSign_Value[]) -> Terminator124/1
  GroundTruth_Access_TrafficSigns/22(TrfSign_Height[m]) -> Terminator125/1
  GroundTruth_Access_TrafficSigns/23(TrfSign_PolyPts_x[m]) -> Terminator120/1
  GroundTruth_Access_TrafficSigns/24(TrfSign_PolyPts_y[m]) -> Terminator122/1
  GroundTruth_Access_TrafficSigns/25(SupplementarySign_Type[]) -> Terminator123/1
  GroundTruth_Access_TrafficSigns/26(SupplementarySign_Actor[]) -> Terminator121/1
  GroundTruth_Access_TrafficSigns/20(TrfSign_Variability[]) -> Terminator117/1
  GroundTruth_Access_TrafficSigns/19(TrfSign_Width[m]) -> Terminator119/1
  GroundTruth_Access_TrafficSigns/18(TrfSign_Length[m]) -> Terminator118/1
  GroundTruth_Access_TrafficSigns/17(TrfSign_Orientation_z[deg]) -> Terminator116/1
  GroundTruth_Access_TrafficSigns/16(TrfSign_Orientation_y[deg]) -> Terminator127/1
  GroundTruth_Access_TrafficSigns/15(TrfSign_Orientation_x[deg]) -> Terminator126/1
  GroundTruth_Access_TrafficSigns/27(SupplementarySign_Variability[]) -> Terminator129/1
  GroundTruth_Access_TrafficSigns/28(SupplementarySign_Value[]) -> Terminator130/1
  GroundTruth_Access_TrafficSigns/29(SupplementarySign_Value_Unit[]) -> Terminator128/1
  GroundTruth_Access_TrafficSigns/33(SupplementarySign_DirectionArrow_2[]) -> Terminator133/1
  GroundTruth_Access_TrafficSigns/32(SupplementarySign_DirectionArrow_1[]) -> Terminator131/1
  GroundTruth_Access_TrafficSigns/31(SupplementarySign_Num_DirectionArrows[]) -> Terminator136/1
  GroundTruth_Access_TrafficSigns/30(SupplementarySign_Num_AssignedLanes[]) -> Terminator135/1
  Enable_TrfSigns_Access[0Off|1On]/1 -> GroundTruth_Access_TrafficSigns/1(Enable[0Off|1On])
  Filter_TrfSigns_In_GT_Area[0Off|1On]/1 -> GroundTruth_Access_TrafficSigns/2(Filter_TrfSigns_In_GT_Area[0Off|1On])
  TrfSign_Idx[]/1 -> GroundTruth_Access_TrafficSigns/3(TrfSign_Idx[])
  GroundTruth_Access_TrafficSigns/1(Num_TrfSigns[]) -> Num_TrfSigns[]/1
  GroundTruth_Access_TrafficSigns/2(Num_TrfSigns_in_GT_Area[]) -> Num_TrfSigns_in_GT_Area[]/1
  GroundTruth_Access_StationaryObjects/11(StatObj_Position_z[m]) -> Terminator51/1
  GroundTruth_Access_StationaryObjects/18(StatObj_PolyPts_x[m]) -> Terminator60/1
  GroundTruth_Access_StationaryObjects/4(StatObj_Type[]) -> Terminator44/1
  GroundTruth_Access_StationaryObjects/12(StatObj_Orientation_x[deg]) -> Terminator52/1
  GroundTruth_Access_StationaryObjects/15(StatObj_Length[m]) -> Terminator57/1
  GroundTruth_Access_StationaryObjects/14(StatObj_Orientation_z[deg]) -> Terminator54/1
  GroundTruth_Access_StationaryObjects/8(StatObj_Color[]) -> Terminator48/1
  GroundTruth_Access_StationaryObjects/3(Flag_StatObj_in_GT_Area[]) -> Terminator43/1
  GroundTruth_Access_StationaryObjects/10(StatObj_Position_y[m]) -> Terminator50/1
  GroundTruth_Access_StationaryObjects/7(StatObj_Density[]) -> Terminator47/1
  GroundTruth_Access_StationaryObjects/9(StatObj_Position_x[m]) -> Terminator49/1
  GroundTruth_Access_StationaryObjects/6(StatObj_Material[]) -> Terminator46/1
  GroundTruth_Access_StationaryObjects/13(StatObj_Orientation_y[deg]) -> Terminator53/1
  GroundTruth_Access_StationaryObjects/16(StatObj_Width[m]) -> Terminator58/1
  GroundTruth_Access_StationaryObjects/19(StatObj_PolyPts_y[m]) -> Terminator61/1
  GroundTruth_Access_StationaryObjects/17(StatObj_Height[m]) -> Terminator59/1
  GroundTruth_Access_StationaryObjects/5(StatObj_ID[]) -> Terminator45/1
  GroundTruth_Access_StationaryObjects/1(Num_StatObj[]) -> Num_StatObj[]/1
